simulink model "NBMS_App_Harness1"  (R2026b)
(part 3 of 4)

      AppIn_G3CommonFlt = false;
      state step_4_1
        AppIn_PMosfetfb = true;
      state step_4_2
        AppIn_HVMosfetfb = true;
      state step_4_3
        AppIn_DCDCMosfetfb = true;
      state step_4_4
        AppIn_PMosfetfb = false;
      (default) -> SleepToDischgToFlt2.step_4.step_4_1
      SleepToDischgToFlt2.step_4.step_4_1 -> SleepToDischgToFlt2.step_4.step_4_2 : [
          | after(0.2,sec)
          | ]
      SleepToDischgToFlt2.step_4.step_4_2 -> SleepToDischgToFlt2.step_4.step_4_3 : [
          | after(0.2,sec)
          | ]
      SleepToDischgToFlt2.step_4.step_4_3 -> SleepToDischgToFlt2.step_4.step_4_4 : [
          | after(0.2,sec)
          | ]
    state step_5
      AppIn_HardwiredIgn = false;
      state step_5_1
        AppIn_HVMosfetfb = false;
      (default) -> SleepToDischgToFlt2.step_5.step_5_1
    SleepToDischgToFlt2.step_6 -> SleepToDischgToFlt2.step_4 : [
        | after(0.2,sec)
        | ]
    (default) -> SleepToDischgToFlt2.Run
    SleepToDischgToFlt2.Run -> SleepToDischgToFlt2.step_1
    SleepToDischgToFlt2.step_1 -> SleepToDischgToFlt2.step_2 : [
        | after(0.2,sec)
        | ]
    SleepToDischgToFlt2.step_2 -> SleepToDischgToFlt2.step_3 : [
        | after(2,sec)
        | ]
    SleepToDischgToFlt2.step_3 -> SleepToDischgToFlt2.step_6 : [
        | after(6,sec)
        | ]
    SleepToDischgToFlt2.step_4 -> SleepToDischgToFlt2.step_5 : [
        | after(2,sec)
        | ]
  state SleepToDischgToFlt3
    state Run
      %% Initialize data outputs.
      AppIn_HardwiredIgn = false;
      AppIn_OBCwakeup = OBC_E.Sleep;
      AppIn_RTCwakeup = false;
      AppIn_MCUHVIL = false;
      AppIn_OBCHVIL = false;
      AppIn_SoCLEDSW = false;
      AppIn_ChgMode = Charger_Mode_E.OFF;
      AppIn_CVmodeTimer = CV_Mode_Timer_E.Off;
      AppIn_TRerror = false;
      AppIn_TRtimer = false;
      AppIn_G3CommonFlt = false;
      AppIn_G3DischargeFlt = false;
      AppIn_G4T1DischargeFlt = false;
      AppIn_G4T2DischargeFlt = false;
      AppIn_G4CommonFlt = false;
      AppIn_G4ChargeFlt = false;
      AppIn_OBCHeartbeatFail = false;
      AppIn_LoadVolt = 63;
      AppIn_PackVolt = 64;
      AppIn_ActiveDischg = Active_DisChrg_E.Inactive;
      AppIn_BattTemp = [26; 26; 26; 26; 26; 26;];
      AppIn_BattCurrent = 0;
      AppIn_BattVoltages = [4.2; 4.2; 4.2; 4.2; 4.2; 4.2; 4.2; 4.2; 4.2; 4.2; 4.2; 4.2; 4.2; 4.2; 4.2; 4.2; 4.2; 4.2; 4.2; 4.2];
      AppIn_LastStoredSOC = 0;
      AppIn_LastStoredCycle = 0;
      AppIn_I2Cerror = false;
      AppIn_LastStoredSOH = 0;
      AppIn_MachineStatus = VDU_MACHINE_STS_E.VDU_SLEEP;
      AppIn_HVMosfetfb = false;
      AppIn_DCDCMosfetfb = false;
      AppIn_PMosfetfb = false;
      AppIn_BMSVltSnsrFail = false;
      AppIn_BattPackTempSnsrFail = false;
      AppIn_VltImbFlt = false;
      AppIn_TempImbWarn = false;
      AppIn_EEPROMSoCWarn15 = false;
    state step_1
      AppIn_HardwiredIgn = true;
    state step_2
      AppIn_MCUHVIL = true;
      state step_2_1
        AppIn_PMosfetfb = true;
      state step_2_2
        AppIn_HVMosfetfb = true;
      state step_2_3
        AppIn_DCDCMosfetfb = true;
      state step_2_4
        AppIn_PMosfetfb = false;
      (default) -> SleepToDischgToFlt3.step_2.step_2_1
      SleepToDischgToFlt3.step_2.step_2_1 -> SleepToDischgToFlt3.step_2.step_2_2 : [
          | after(0.2,sec)
          | ]
      SleepToDischgToFlt3.step_2.step_2_2 -> SleepToDischgToFlt3.step_2.step_2_3 : [
          | after(0.2,sec)
          | ]
      SleepToDischgToFlt3.step_2.step_2_3 -> SleepToDischgToFlt3.step_2.step_2_4 : [
          | after(0.2,sec)
          | ]
    state step_3
      AppIn_G4CommonFlt = true;
    state step_6
      AppIn_OBCHVIL = true;
    state step_4
      AppIn_OBCHVIL = false;
      AppIn_G4CommonFlt = false;
      state step_4_1
        AppIn_PMosfetfb = true;
      state step_4_2
        AppIn_HVMosfetfb = true;
      state step_4_3
        AppIn_DCDCMosfetfb = true;
      state step_4_4
        AppIn_PMosfetfb = false;
      (default) -> SleepToDischgToFlt3.step_4.step_4_1
      SleepToDischgToFlt3.step_4.step_4_1 -> SleepToDischgToFlt3.step_4.step_4_2 : [
          | after(0.2,sec)
          | ]
      SleepToDischgToFlt3.step_4.step_4_2 -> SleepToDischgToFlt3.step_4.step_4_3 : [
          | after(0.2,sec)
          | ]
      SleepToDischgToFlt3.step_4.step_4_3 -> SleepToDischgToFlt3.step_4.step_4_4 : [
          | after(0.2,sec)
          | ]
    state step_5
      AppIn_HardwiredIgn = false;
      state step_5_1
        AppIn_HVMosfetfb = false;
      (default) -> SleepToDischgToFlt3.step_5.step_5_1
    (default) -> SleepToDischgToFlt3.Run
    SleepToDischgToFlt3.Run -> SleepToDischgToFlt3.step_1
    SleepToDischgToFlt3.step_1 -> SleepToDischgToFlt3.step_2 : [
        | after(0.2,sec)
        | ]
    SleepToDischgToFlt3.step_2 -> SleepToDischgToFlt3.step_3 : [
        | after(2,sec)
        | ]
    SleepToDischgToFlt3.step_3 -> SleepToDischgToFlt3.step_6 : [
        | after(6,sec)
        | ]
    SleepToDischgToFlt3.step_6 -> SleepToDischgToFlt3.step_4 : [
        | after(0.2,sec)
        | ]
    SleepToDischgToFlt3.step_4 -> SleepToDischgToFlt3.step_5 : [
        | after(2,sec)
        | ]
  state SleepToChgToFlt
    state Run
      %% Initialize data outputs.
      AppIn_HardwiredIgn = false;
      AppIn_OBCwakeup = OBC_E.Sleep;
      AppIn_RTCwakeup = false;
      AppIn_MCUHVIL = false;
      AppIn_OBCHVIL = false;
      AppIn_SoCLEDSW = false;
      AppIn_ChgMode = Charger_Mode_E.OFF;
      AppIn_CVmodeTimer = CV_Mode_Timer_E.Off;
      AppIn_TRerror = false;
      AppIn_TRtimer = false;
      AppIn_G3CommonFlt = false;
      AppIn_G3DischargeFlt = false;
      AppIn_G4T1DischargeFlt = false;
      AppIn_G4T2DischargeFlt = false;
      AppIn_G4CommonFlt = false;
      AppIn_G4ChargeFlt = false;
      AppIn_OBCHeartbeatFail = false;
      AppIn_LoadVolt = 63;
      AppIn_PackVolt = 64;
      AppIn_ActiveDischg = Active_DisChrg_E.Inactive;
      AppIn_BattTemp = [26; 26; 26; 26; 26; 26;];
      AppIn_BattCurrent = 0;
      AppIn_BattVoltages = [4.2; 4.2; 4.2; 4.2; 4.2; 4.2; 4.2; 4.2; 4.2; 4.2; 4.2; 4.2; 4.2; 4.2; 4.2; 4.2; 4.2; 4.2; 4.2; 4.2];
      AppIn_LastStoredSOC = 0;
      AppIn_LastStoredCycle = 0;
      AppIn_I2Cerror = false;
      AppIn_LastStoredSOH = 0;
      AppIn_MachineStatus = VDU_MACHINE_STS_E.VDU_SLEEP;
      AppIn_HVMosfetfb = false;
      AppIn_DCDCMosfetfb = false;
      AppIn_PMosfetfb = false;
      AppIn_BMSVltSnsrFail = false;
      AppIn_BattPackTempSnsrFail = false;
      AppIn_VltImbFlt = false;
      AppIn_TempImbWarn = false;
      AppIn_EEPROMSoCWarn15 = false;
    state step_1
      AppIn_OBCwakeup = OBC_E.Wake_Up;
      AppIn_OBCHVIL = true;
    state step_2
      state step_2_1
        AppIn_PMosfetfb = true;
      state step_2_2
        AppIn_HVMosfetfb = true;
      state step_2_3
        AppIn_PMosfetfb = false;
      (default) -> SleepToChgToFlt.step_2.step_2_1
      SleepToChgToFlt.step_2.step_2_1 -> SleepToChgToFlt.step_2.step_2_2 : [
          | after(0.3,sec)
          | ]
      SleepToChgToFlt.step_2.step_2_2 -> SleepToChgToFlt.step_2.step_2_3 : [
          | after(0.5,sec)
          | ]
    state step_3
      AppIn_G3CommonFlt = true;
    state step_4
      state step_4_1
        AppIn_ChgMode = Charger_Mode_E.Error;
      state step_4_2
        AppIn_ChgMode = Charger_Mode_E.OFF;
      (default) -> SleepToChgToFlt.step_4.step_4_1
      SleepToChgToFlt.step_4.step_4_1 -> SleepToChgToFlt.step_4.step_4_2 : [
          | after(0.1,sec)
          | ]
    state step_5
      AppIn_G3CommonFlt = false;
    state step_6
      AppIn_OBCHVIL = false;
      AppIn_OBCwakeup = OBC_E.Sleep;
      state step_6_1
        AppIn_HVMosfetfb = false;
      (default) -> SleepToChgToFlt.step_6.step_6_1
    (default) -> SleepToChgToFlt.Run
    SleepToChgToFlt.Run -> SleepToChgToFlt.step_1 : [
        | after(0.2,sec)
        | ]
    SleepToChgToFlt.step_1 -> SleepToChgToFlt.step_2 : [
        | after(0.2,sec)
        | ]
    SleepToChgToFlt.step_2 -> SleepToChgToFlt.step_3 : [
        | after(2,sec)
        | ]
    SleepToChgToFlt.step_3 -> SleepToChgToFlt.step_4 : [
        | after(1,sec)
        | ]
    SleepToChgToFlt.step_4 -> SleepToChgToFlt.step_5 : [
        | after(1,sec)
        | ]
    SleepToChgToFlt.step_5 -> SleepToChgToFlt.step_6 : [
        | after(2,sec)
        | ]
  state SleepToChgToFltToDischg
    state Run
      %% Initialize data outputs.
      AppIn_HardwiredIgn = false;
      AppIn_OBCwakeup = OBC_E.Sleep;
      AppIn_RTCwakeup = false;
      AppIn_MCUHVIL = false;
      AppIn_OBCHVIL = false;
      AppIn_SoCLEDSW = false;
      AppIn_ChgMode = Charger_Mode_E.OFF;
      AppIn_CVmodeTimer = CV_Mode_Timer_E.Off;
      AppIn_TRerror = false;
      AppIn_TRtimer = false;
      AppIn_G3CommonFlt = false;
      AppIn_G3DischargeFlt = false;
      AppIn_G4T1DischargeFlt = false;
      AppIn_G4T2DischargeFlt = false;
      AppIn_G4CommonFlt = false;
      AppIn_G4ChargeFlt = false;
      AppIn_OBCHeartbeatFail = false;
      AppIn_LoadVolt = 63;
      AppIn_PackVolt = 64;
      AppIn_ActiveDischg = Active_DisChrg_E.Inactive;
      AppIn_BattTemp = [26; 26; 26; 26; 26; 26;];
      AppIn_BattCurrent = 0;
      AppIn_BattVoltages = [4.2; 4.2; 4.2; 4.2; 4.2; 4.2; 4.2; 4.2; 4.2; 4.2; 4.2; 4.2; 4.2; 4.2; 4.2; 4.2; 4.2; 4.2; 4.2; 4.2];
      AppIn_LastStoredSOC = 0;
      AppIn_LastStoredCycle = 0;
      AppIn_I2Cerror = false;
      AppIn_LastStoredSOH = 0;
      AppIn_MachineStatus = VDU_MACHINE_STS_E.VDU_SLEEP;
      AppIn_HVMosfetfb = false;
      AppIn_DCDCMosfetfb = false;
      AppIn_PMosfetfb = false;
      AppIn_BMSVltSnsrFail = false;
      AppIn_BattPackTempSnsrFail = false;
      AppIn_VltImbFlt = false;
      AppIn_TempImbWarn = false;
      AppIn_EEPROMSoCWarn15 = false;
    state step_1
      AppIn_OBCwakeup = OBC_E.Wake_Up;
      AppIn_OBCHVIL = true;
    state step_2
      state step_2_1
        AppIn_PMosfetfb = true;
      state step_2_2
        AppIn_HVMosfetfb = true;
      state step_2_3
        AppIn_PMosfetfb = false;
      (default) -> SleepToChgToFltToDischg.step_2.step_2_1
      SleepToChgToFltToDischg.step_2.step_2_1 -> SleepToChgToFltToDischg.step_2.step_2_2 : [
          | after(0.3,sec)
          | ]
      SleepToChgToFltToDischg.step_2.step_2_2 -> SleepToChgToFltToDischg.step_2.step_2_3 : [
          | after(0.5,sec)
          | ]
    state step_3
      AppIn_G4ChargeFlt= true;
    state step_4
      AppIn_OBCHVIL = false;
      AppIn_OBCwakeup = OBC_E.Sleep;
      AppIn_HardwiredIgn = true;
      AppIn_MCUHVIL = true;
      state step_4_1
        AppIn_PMosfetfb = true;
      state step_4_2
        AppIn_HVMosfetfb = true;
      state step_4_3
        AppIn_DCDCMosfetfb = true;
      state step_4_4
        AppIn_PMosfetfb = false;
      (default) -> SleepToChgToFltToDischg.step_4.step_4_1
      SleepToChgToFltToDischg.step_4.step_4_1 -> SleepToChgToFltToDischg.step_4.step_4_2 : [
          | after(0.3,sec)
          | ]
      SleepToChgToFltToDischg.step_4.step_4_2 -> SleepToChgToFltToDischg.step_4.step_4_3 : [
          | after(0.2,sec)
          | ]
      SleepToChgToFltToDischg.step_4.step_4_3 -> SleepToChgToFltToDischg.step_4.step_4_4 : [
          | after(0.2,sec)
          | ]
    state step_5
      AppIn_HardwiredIgn = false;
      state step_6_1
        AppIn_HVMosfetfb = false;
      (default) -> SleepToChgToFltToDischg.step_5.step_6_1
    (default) -> SleepToChgToFltToDischg.Run
    SleepToChgToFltToDischg.Run -> SleepToChgToFltToDischg.step_1 : [
        | after(0.2,sec)
        | ]
    SleepToChgToFltToDischg.step_1 -> SleepToChgToFltToDischg.step_2 : [
        | after(0.2,sec)
        | ]
    SleepToChgToFltToDischg.step_2 -> SleepToChgToFltToDischg.step_3 : [
        | after(2,sec)
        | ]
    SleepToChgToFltToDischg.step_3 -> SleepToChgToFltToDischg.step_4 : [
        | after(1,sec)
        | ]
    SleepToChgToFltToDischg.step_4 -> SleepToChgToFltToDischg.step_5 : [
        | after(2,sec)
        | ]
  state SleepToChgToFltToDischg1
    state Run
      %% Initialize data outputs.
      AppIn_HardwiredIgn = false;
      AppIn_OBCwakeup = OBC_E.Sleep;
      AppIn_RTCwakeup = false;
      AppIn_MCUHVIL = false;
      AppIn_OBCHVIL = false;
      AppIn_SoCLEDSW = false;
      AppIn_ChgMode = Charger_Mode_E.OFF;
      AppIn_CVmodeTimer = CV_Mode_Timer_E.Off;
      AppIn_TRerror = false;
      AppIn_TRtimer = false;
      AppIn_G3CommonFlt = false;
      AppIn_G3DischargeFlt = false;
      AppIn_G4T1DischargeFlt = false;
      AppIn_G4T2DischargeFlt = false;
      AppIn_G4CommonFlt = false;
      AppIn_G4ChargeFlt = false;
      AppIn_OBCHeartbeatFail = false;
      AppIn_LoadVolt = 63;
      AppIn_PackVolt = 64;
      AppIn_ActiveDischg = Active_DisChrg_E.Inactive;
      AppIn_BattTemp = [26; 26; 26; 26; 26; 26;];
      AppIn_BattCurrent = 0;
      AppIn_BattVoltages = [4.2; 4.2; 4.2; 4.2; 4.2; 4.2; 4.2; 4.2; 4.2; 4.2; 4.2; 4.2; 4.2; 4.2; 4.2; 4.2; 4.2; 4.2; 4.2; 4.2];
      AppIn_LastStoredSOC = 0;
      AppIn_LastStoredCycle = 0;
      AppIn_I2Cerror = false;
      AppIn_LastStoredSOH = 0;
      AppIn_MachineStatus = VDU_MACHINE_STS_E.VDU_SLEEP;
      AppIn_HVMosfetfb = false;
      AppIn_DCDCMosfetfb = false;
      AppIn_PMosfetfb = false;
      AppIn_BMSVltSnsrFail = false;
      AppIn_BattPackTempSnsrFail = false;
      AppIn_VltImbFlt = false;
      AppIn_TempImbWarn = false;
      AppIn_EEPROMSoCWarn15 = false;
    state step_1
      AppIn_OBCwakeup = OBC_E.Wake_Up;
      AppIn_OBCHVIL = true;
    state step_2
      state step_2_1
        AppIn_PMosfetfb = true;
      state step_2_2
        AppIn_HVMosfetfb = true;
      state step_2_3
        AppIn_PMosfetfb = false;
      (default) -> SleepToChgToFltToDischg1.step_2.step_2_1
      SleepToChgToFltToDischg1.step_2.step_2_1 -> SleepToChgToFltToDischg1.step_2.step_2_2 : [
          | after(0.3,sec)
          | ]
      SleepToChgToFltToDischg1.step_2.step_2_2 -> SleepToChgToFltToDischg1.step_2.step_2_3 : [
          | after(0.5,sec)
          | ]
    state step_3
      AppIn_G4CommonFlt= true;
    state step_4
      AppIn_OBCHVIL = false;
      AppIn_OBCwakeup = OBC_E.Sleep;
      AppIn_HardwiredIgn = true;
      AppIn_MCUHVIL = true;
      AppIn_G4CommonFlt= false;
      state step_4_1
        AppIn_PMosfetfb = true;
      state step_4_2
        AppIn_HVMosfetfb = true;
      state step_4_3
        AppIn_DCDCMosfetfb = true;
      state step_4_4
        AppIn_PMosfetfb = false;
      (default) -> SleepToChgToFltToDischg1.step_4.step_4_1
      SleepToChgToFltToDischg1.step_4.step_4_1 -> SleepToChgToFltToDischg1.step_4.step_4_2 : [
          | after(0.3,sec)
          | ]
      SleepToChgToFltToDischg1.step_4.step_4_2 -> SleepToChgToFltToDischg1.step_4.step_4_3 : [
          | after(0.2,sec)
          | ]
      SleepToChgToFltToDischg1.step_4.step_4_3 -> SleepToChgToFltToDischg1.step_4.step_4_4 : [
          | after(0.2,sec)
          | ]
    state step_5
      AppIn_HardwiredIgn = false;
      state step_6_1
        AppIn_HVMosfetfb = false;
      (default) -> SleepToChgToFltToDischg1.step_5.step_6_1
    state step_6
      AppIn_G4CommonFlt= true;
    (default) -> SleepToChgToFltToDischg1.Run
    SleepToChgToFltToDischg1.Run -> SleepToChgToFltToDischg1.step_1 : [
        | after(0.2,sec)
        | ]
    SleepToChgToFltToDischg1.step_1 -> SleepToChgToFltToDischg1.step_2 : [
        | after(0.2,sec)
        | ]
    SleepToChgToFltToDischg1.step_2 -> SleepToChgToFltToDischg1.step_3 : [
        | after(2,sec)
        | ]
    SleepToChgToFltToDischg1.step_3 -> SleepToChgToFltToDischg1.step_4 : [
        | after(1,sec)
        | ]
    SleepToChgToFltToDischg1.step_4 -> SleepToChgToFltToDischg1.step_5 : [
        | after(2,sec)
        | ]
    SleepToChgToFltToDischg1.step_5 -> SleepToChgToFltToDischg1.step_6 : [
        | after(0.3,sec)
        | ]
  state SleepToDischgToFltToChg
    state Run
      %% Initialize data outputs.
      AppIn_HardwiredIgn = false;
      AppIn_OBCwakeup = OBC_E.Sleep;
      AppIn_RTCwakeup = false;
      AppIn_MCUHVIL = false;
      AppIn_OBCHVIL = false;
      AppIn_SoCLEDSW = false;
      AppIn_ChgMode = Charger_Mode_E.OFF;
      AppIn_CVmodeTimer = CV_Mode_Timer_E.Off;
      AppIn_TRerror = false;
      AppIn_TRtimer = false;
      AppIn_G3CommonFlt = false;
      AppIn_G3DischargeFlt = false;
      AppIn_G4T1DischargeFlt = false;
      AppIn_G4T2DischargeFlt = false;
      AppIn_G4CommonFlt = false;
      AppIn_G4ChargeFlt = false;
      AppIn_OBCHeartbeatFail = false;
      AppIn_LoadVolt = 63;
      AppIn_PackVolt = 64;
      AppIn_ActiveDischg = Active_DisChrg_E.Inactive;
      AppIn_BattTemp = [26; 26; 26; 26; 26; 26;];
      AppIn_BattCurrent = 0;
      AppIn_BattVoltages = [4.2; 4.2; 4.2; 4.2; 4.2; 4.2; 4.2; 4.2; 4.2; 4.2; 4.2; 4.2; 4.2; 4.2; 4.2; 4.2; 4.2; 4.2; 4.2; 4.2];
      AppIn_LastStoredSOC = 0;
      AppIn_LastStoredCycle = 0;
      AppIn_I2Cerror = false;
      AppIn_LastStoredSOH = 0;
      AppIn_MachineStatus = VDU_MACHINE_STS_E.VDU_SLEEP;
      AppIn_HVMosfetfb = false;
      AppIn_DCDCMosfetfb = false;
      AppIn_PMosfetfb = false;
      AppIn_BMSVltSnsrFail = false;
      AppIn_BattPackTempSnsrFail = false;
      AppIn_VltImbFlt = false;
      AppIn_TempImbWarn = false;
      AppIn_EEPROMSoCWarn15 = false;
    state step_1
      AppIn_HardwiredIgn = true;
      AppIn_MCUHVIL = true;
    state step_2
      state step_2_1
        AppIn_PMosfetfb = true;
      state step_2_2
        AppIn_HVMosfetfb = true;
      state step_2_4
        AppIn_DCDCMosfetfb = true;
      state step_2_3
        AppIn_PMosfetfb = false;
      (default) -> SleepToDischgToFltToChg.step_2.step_2_1
      SleepToDischgToFltToChg.step_2.step_2_1 -> SleepToDischgToFltToChg.step_2.step_2_2 : [
          | after(0.3,sec)
          | ]
      SleepToDischgToFltToChg.step_2.step_2_2 -> SleepToDischgToFltToChg.step_2.step_2_4 : [
          | after(0.2,sec)
          | ]
      SleepToDischgToFltToChg.step_2.step_2_4 -> SleepToDischgToFltToChg.step_2.step_2_3 : [
          | after(0.2,sec)
          | ]
    state step_3
      AppIn_G4T1DischargeFlt= true;
    state step_4
      AppIn_OBCHVIL = true;
      AppIn_OBCwakeup = OBC_E.Wake_Up;
      state step_4_1
        AppIn_PMosfetfb = true;
      state step_4_2
        AppIn_HVMosfetfb = true;
      state step_4_3
        AppIn_DCDCMosfetfb = true;
      state step_4_4
        AppIn_PMosfetfb = false;
      (default) -> SleepToDischgToFltToChg.step_4.step_4_1
      SleepToDischgToFltToChg.step_4.step_4_1 -> SleepToDischgToFltToChg.step_4.step_4_2 : [
          | after(0.3,sec)
          | ]
      SleepToDischgToFltToChg.step_4.step_4_2 -> SleepToDischgToFltToChg.step_4.step_4_3 : [
          | after(0.2,sec)
          | ]
      SleepToDischgToFltToChg.step_4.step_4_3 -> SleepToDischgToFltToChg.step_4.step_4_4 : [
          | after(0.2,sec)
          | ]
    state step_5
      AppIn_HardwiredIgn = false;
      AppIn_OBCHVIL = false;
      AppIn_OBCwakeup = OBC_E.Sleep;
      state step_6_1
        AppIn_HVMosfetfb = false;
      (default) -> SleepToDischgToFltToChg.step_5.step_6_1
    (default) -> SleepToDischgToFltToChg.Run
    SleepToDischgToFltToChg.Run -> SleepToDischgToFltToChg.step_1 : [
        | after(0.2,sec)
        | ]
    SleepToDischgToFltToChg.step_1 -> SleepToDischgToFltToChg.step_2 : [
        | after(0.2,sec)
        | ]
    SleepToDischgToFltToChg.step_2 -> SleepToDischgToFltToChg.step_3 : [
        | after(2,sec)
        | ]
    SleepToDischgToFltToChg.step_3 -> SleepToDischgToFltToChg.step_4 : [
        | after(1,sec)
        | ]
    SleepToDischgToFltToChg.step_4 -> SleepToDischgToFltToChg.step_5 : [
        | after(2,sec)
        | ]
  state SleepToDischgToFltToChg1
    state Run
      %% Initialize data outputs.
      AppIn_HardwiredIgn = false;
      AppIn_OBCwakeup = OBC_E.Sleep;
      AppIn_RTCwakeup = false;
      AppIn_MCUHVIL = false;
      AppIn_OBCHVIL = false;
      AppIn_SoCLEDSW = false;
      AppIn_ChgMode = Charger_Mode_E.OFF;
      AppIn_CVmodeTimer = CV_Mode_Timer_E.Off;
      AppIn_TRerror = false;
      AppIn_TRtimer = false;
      AppIn_G3CommonFlt = false;
      AppIn_G3DischargeFlt = false;
      AppIn_G4T1DischargeFlt = false;
      AppIn_G4T2DischargeFlt = false;
      AppIn_G4CommonFlt = false;
      AppIn_G4ChargeFlt = false;
      AppIn_OBCHeartbeatFail = false;
      AppIn_LoadVolt = 63;
      AppIn_PackVolt = 64;
      AppIn_ActiveDischg = Active_DisChrg_E.Inactive;
      AppIn_BattTemp = [26; 26; 26; 26; 26; 26;];
      AppIn_BattCurrent = 0;
      AppIn_BattVoltages = [4.2; 4.2; 4.2; 4.2; 4.2; 4.2; 4.2; 4.2; 4.2; 4.2; 4.2; 4.2; 4.2; 4.2; 4.2; 4.2; 4.2; 4.2; 4.2; 4.2];
      AppIn_LastStoredSOC = 0;
      AppIn_LastStoredCycle = 0;
      AppIn_I2Cerror = false;
      AppIn_LastStoredSOH = 0;
      AppIn_MachineStatus = VDU_MACHINE_STS_E.VDU_SLEEP;
      AppIn_HVMosfetfb = false;
      AppIn_DCDCMosfetfb = false;
      AppIn_PMosfetfb = false;
      AppIn_BMSVltSnsrFail = false;
      AppIn_BattPackTempSnsrFail = false;
      AppIn_VltImbFlt = false;
      AppIn_TempImbWarn = false;
      AppIn_EEPROMSoCWarn15 = false;
    state step_1
      AppIn_HardwiredIgn = true;
      AppIn_MCUHVIL = true;
    state step_2
      state step_2_1
        AppIn_PMosfetfb = true;
      state step_2_2
        AppIn_HVMosfetfb = true;
      state step_2_4
        AppIn_DCDCMosfetfb = true;
      state step_2_3
        AppIn_PMosfetfb = false;
      (default) -> SleepToDischgToFltToChg1.step_2.step_2_1
      SleepToDischgToFltToChg1.step_2.step_2_1 -> SleepToDischgToFltToChg1.step_2.step_2_2 : [
          | after(0.3,sec)
          | ]
      SleepToDischgToFltToChg1.step_2.step_2_2 -> SleepToDischgToFltToChg1.step_2.step_2_4 : [
          | after(0.2,sec)
          | ]
      SleepToDischgToFltToChg1.step_2.step_2_4 -> SleepToDischgToFltToChg1.step_2.step_2_3 : [
          | after(0.2,sec)
          | ]
    state step_3
      AppIn_G3DischargeFlt= true;
    state step_4
      AppIn_OBCHVIL = true;
      AppIn_OBCwakeup = OBC_E.Wake_Up;
      state step_4_1
        AppIn_PMosfetfb = true;
      state step_4_2
        AppIn_HVMosfetfb = true;
      state step_4_3
        AppIn_DCDCMosfetfb = true;
      state step_4_4
        AppIn_PMosfetfb = false;
      (default) -> SleepToDischgToFltToChg1.step_4.step_4_1
      SleepToDischgToFltToChg1.step_4.step_4_1 -> SleepToDischgToFltToChg1.step_4.step_4_2 : [
          | after(0.3,sec)
          | ]
      SleepToDischgToFltToChg1.step_4.step_4_2 -> SleepToDischgToFltToChg1.step_4.step_4_3 : [
          | after(0.2,sec)
          | ]
      SleepToDischgToFltToChg1.step_4.step_4_3 -> SleepToDischgToFltToChg1.step_4.step_4_4 : [
          | after(0.2,sec)
          | ]
    state step_5
      AppIn_HardwiredIgn = false;
      AppIn_OBCHVIL = false;
      AppIn_OBCwakeup = OBC_E.Sleep;
      state step_6_1
        AppIn_HVMosfetfb = false;
      (default) -> SleepToDischgToFltToChg1.step_5.step_6_1
    (default) -> SleepToDischgToFltToChg1.Run
    SleepToDischgToFltToChg1.Run -> SleepToDischgToFltToChg1.step_1 : [
        | after(0.2,sec)
        | ]
    SleepToDischgToFltToChg1.step_1 -> SleepToDischgToFltToChg1.step_2 : [
        | after(0.2,sec)
        | ]
    SleepToDischgToFltToChg1.step_2 -> SleepToDischgToFltToChg1.step_3 : [
        | after(2,sec)
        | ]
    SleepToDischgToFltToChg1.step_3 -> SleepToDischgToFltToChg1.step_4 : [
        | after(1,sec)
        | ]
    SleepToDischgToFltToChg1.step_4 -> SleepToDischgToFltToChg1.step_5 : [
        | after(2,sec)
        | ]
  state SleepToDischgToFltToChg2
    state Run
      %% Initialize data outputs.
      AppIn_HardwiredIgn = false;
      AppIn_OBCwakeup = OBC_E.Sleep;
      AppIn_RTCwakeup = false;
      AppIn_MCUHVIL = false;
      AppIn_OBCHVIL = false;
      AppIn_SoCLEDSW = false;
      AppIn_ChgMode = Charger_Mode_E.OFF;
      AppIn_CVmodeTimer = CV_Mode_Timer_E.Off;
      AppIn_TRerror = false;
      AppIn_TRtimer = false;
      AppIn_G3CommonFlt = false;
      AppIn_G3DischargeFlt = false;
      AppIn_G4T1DischargeFlt = false;
      AppIn_G4T2DischargeFlt = false;
      AppIn_G4CommonFlt = false;
      AppIn_G4ChargeFlt = false;
      AppIn_OBCHeartbeatFail = false;
      AppIn_LoadVolt = 63;
      AppIn_PackVolt = 64;
      AppIn_ActiveDischg = Active_DisChrg_E.Inactive;
      AppIn_BattTemp = [26; 26; 26; 26; 26; 26;];
      AppIn_BattCurrent = 0;
      AppIn_BattVoltages = [4.2; 4.2; 4.2; 4.2; 4.2; 4.2; 4.2; 4.2; 4.2; 4.2; 4.2; 4.2; 4.2; 4.2; 4.2; 4.2; 4.2; 4.2; 4.2; 4.2];
      AppIn_LastStoredSOC = 0;
      AppIn_LastStoredCycle = 0;
      AppIn_I2Cerror = false;
      AppIn_LastStoredSOH = 0;
      AppIn_MachineStatus = VDU_MACHINE_STS_E.VDU_SLEEP;
      AppIn_HVMosfetfb = false;
      AppIn_DCDCMosfetfb = false;
      AppIn_PMosfetfb = false;
      AppIn_BMSVltSnsrFail = false;
      AppIn_BattPackTempSnsrFail = false;
      AppIn_VltImbFlt = false;
      AppIn_TempImbWarn = false;
      AppIn_EEPROMSoCWarn15 = false;
    state step_1
      AppIn_HardwiredIgn = true;
      AppIn_MCUHVIL = true;
    state step_2
      state step_2_1
        AppIn_PMosfetfb = true;
      state step_2_2
        AppIn_HVMosfetfb = true;
      state step_2_4
        AppIn_DCDCMosfetfb = true;
      state step_2_3
        AppIn_PMosfetfb = false;
      (default) -> SleepToDischgToFltToChg2.step_2.step_2_1
      SleepToDischgToFltToChg2.step_2.step_2_1 -> SleepToDischgToFltToChg2.step_2.step_2_2 : [
          | after(0.3,sec)
          | ]
      SleepToDischgToFltToChg2.step_2.step_2_2 -> SleepToDischgToFltToChg2.step_2.step_2_4 : [
          | after(0.2,sec)
          | ]
      SleepToDischgToFltToChg2.step_2.step_2_4 -> SleepToDischgToFltToChg2.step_2.step_2_3 : [
          | after(0.2,sec)
          | ]
    state step_3
      AppIn_G4T2DischargeFlt= true;
    state step_4
      AppIn_OBCHVIL = true;
      AppIn_OBCwakeup = OBC_E.Wake_Up;
      state step_4_1
        AppIn_PMosfetfb = true;
      state step_4_2
        AppIn_HVMosfetfb = true;
      state step_4_3
        AppIn_DCDCMosfetfb = true;
      state step_4_4
        AppIn_PMosfetfb = false;
      (default) -> SleepToDischgToFltToChg2.step_4.step_4_1
      SleepToDischgToFltToChg2.step_4.step_4_1 -> SleepToDischgToFltToChg2.step_4.step_4_2 : [
          | after(0.3,sec)
          | ]
      SleepToDischgToFltToChg2.step_4.step_4_2 -> SleepToDischgToFltToChg2.step_4.step_4_3 : [
          | after(0.2,sec)
          | ]
      SleepToDischgToFltToChg2.step_4.step_4_3 -> SleepToDischgToFltToChg2.step_4.step_4_4 : [
          | after(0.2,sec)
          | ]
    state step_5
      AppIn_HardwiredIgn = false;
      AppIn_OBCHVIL = false;
      AppIn_OBCwakeup = OBC_E.Sleep;
      state step_6_1
        AppIn_HVMosfetfb = false;
      (default) -> SleepToDischgToFltToChg2.step_5.step_6_1
    (default) -> SleepToDischgToFltToChg2.Run
    SleepToDischgToFltToChg2.Run -> SleepToDischgToFltToChg2.step_1 : [
        | after(0.2,sec)
        | ]
    SleepToDischgToFltToChg2.step_1 -> SleepToDischgToFltToChg2.step_2 : [
        | after(0.2,sec)
        | ]
    SleepToDischgToFltToChg2.step_2 -> SleepToDischgToFltToChg2.step_3 : [
        | after(2,sec)
        | ]
    SleepToDischgToFltToChg2.step_3 -> SleepToDischgToFltToChg2.step_4 : [
        | after(1,sec)
        | ]
    SleepToDischgToFltToChg2.step_4 -> SleepToDischgToFltToChg2.step_5 : [
        | after(2,sec)
        | ]
  state ChargingSequence
    state Run
      %% Initialize data outputs.
      AppIn_HardwiredIgn = false;
      AppIn_OBCwakeup = OBC_E.Sleep;
      AppIn_RTCwakeup = false;
      AppIn_MCUHVIL = false;
      AppIn_OBCHVIL = false;
      AppIn_SoCLEDSW = false;
      AppIn_ChgMode = Charger_Mode_E.OFF;
      AppIn_CVmodeTimer = CV_Mode_Timer_E.Off;
      AppIn_TRerror = false;
      AppIn_TRtimer = false;
      AppIn_G3CommonFlt = false;
      AppIn_G3DischargeFlt = false;
      AppIn_G4T1DischargeFlt = false;
      AppIn_G4T2DischargeFlt = false;
      AppIn_G4CommonFlt = false;
      AppIn_G4ChargeFlt = false;
      AppIn_OBCHeartbeatFail = false;
      AppIn_LoadVolt = 78;
      AppIn_PackVolt = 74;
      AppIn_ActiveDischg = Active_DisChrg_E.Inactive;
      AppIn_BattTemp = [26; 26; 26; 26; 26; 26;];
      AppIn_BattCurrent = 0;
      AppIn_BattVoltages = [4.41; 4.41; 4.41; 4.41; 4.41; 4.41; 4.41; 4.41; 4.41; 4.41; 4.41; 4.41; 4.41; 4.41; 4.41; 4.41; 4.41; 4.41; 4.41; 3.2];
      AppIn_LastStoredSOC = 0;
      AppIn_LastStoredCycle = 0;
      AppIn_I2Cerror = false;
      AppIn_LastStoredSOH = 0;
      AppIn_MachineStatus = VDU_MACHINE_STS_E.VDU_SLEEP;
      AppIn_HVMosfetfb = false;
      AppIn_DCDCMosfetfb = false;
      AppIn_PMosfetfb = false;
      AppIn_BMSVltSnsrFail = false;
      AppIn_BattPackTempSnsrFail = false;
      AppIn_VltImbFlt = false;
      AppIn_TempImbWarn = false;
      AppIn_EEPROMSoCWarn15 = false;
    state step_1
      AppIn_OBCwakeup = OBC_E.Wake_Up;
      AppIn_OBCHVIL = true;
    state step_2
      state step_2_1
        AppIn_PMosfetfb = true;
      state step_2_2
        AppIn_HVMosfetfb = true;
      state step_2_3
        AppIn_PMosfetfb = false;
      (default) -> ChargingSequence.step_2.step_2_1
      ChargingSequence.step_2.step_2_1 -> ChargingSequence.step_2.step_2_2 : [
          | after(0.3,sec)
          | ]
      ChargingSequence.step_2.step_2_2 -> ChargingSequence.step_2.step_2_3 : [
          | after(0.5,sec)
          | ]
    state step_4
      AppIn_OBCwakeup = OBC_E.Sleep;
      AppIn_HVMosfetfb = false;
    (default) -> ChargingSequence.Run
    ChargingSequence.Run -> ChargingSequence.step_1 : [
        | after(0.1,sec)
        | ]
    ChargingSequence.step_1 -> ChargingSequence.step_2 : [
        | after(0.2,sec)
        | ]
    ChargingSequence.step_2 -> ChargingSequence.step_4 : [
        | after(6,sec)
        | ]
  state ChargeSeq
    state Run
      %% Initialize data outputs.
      AppIn_HardwiredIgn = false;
      AppIn_OBCwakeup = OBC_E.Sleep;
      AppIn_RTCwakeup = false;
      AppIn_MCUHVIL = false;
      AppIn_OBCHVIL = false;
      AppIn_SoCLEDSW = false;
      AppIn_ChgMode = Charger_Mode_E.OFF;
      AppIn_CVmodeTimer = CV_Mode_Timer_E.Off;
      AppIn_TRerror = false;
      AppIn_TRtimer = false;
      AppIn_G3CommonFlt = false;
      AppIn_G3DischargeFlt = false;
      AppIn_G4T1DischargeFlt = false;
      AppIn_G4T2DischargeFlt = false;
      AppIn_G4CommonFlt = false;
      AppIn_G4ChargeFlt = false;
      AppIn_OBCHeartbeatFail = false;
      AppIn_LoadVolt = 80;
      AppIn_PackVolt = 78;
      AppIn_ActiveDischg = Active_DisChrg_E.Inactive;
      AppIn_BattTemp = [26; 26; 26; 26; 26; 26;];
      AppIn_BattCurrent = 0;
      AppIn_BattVoltages = [4.41; 4.41; 4.41; 4.41; 4.41; 4.41; 4.41; 4.41; 4.41; 4.41; 4.41; 4.41; 4.41; 4.41; 4.41; 4.41; 4.41; 4.41; 4.41; 3.2];
      AppIn_LastStoredSOC = 0;
      AppIn_LastStoredCycle = 0;
      AppIn_I2Cerror = false;
      AppIn_LastStoredSOH = 0;
      AppIn_MachineStatus = VDU_MACHINE_STS_E.VDU_SLEEP;
      AppIn_HVMosfetfb = false;
      AppIn_DCDCMosfetfb = false;
      AppIn_PMosfetfb = false;
      AppIn_BMSVltSnsrFail = false;
      AppIn_BattPackTempSnsrFail = false;
      AppIn_VltImbFlt = false;
      AppIn_TempImbWarn = false;
      AppIn_EEPROMSoCWarn15 = false;
    state step_1
      AppIn_OBCwakeup = OBC_E.Wake_Up;
      AppIn_OBCHVIL = true;
    state step_2
      state step_2_1
        AppIn_PMosfetfb = true;
      state step_2_2
        AppIn_HVMosfetfb = true;
      state step_2_3
        AppIn_PMosfetfb = false;
      (default) -> ChargeSeq.step_2.step_2_1
      ChargeSeq.step_2.step_2_1 -> ChargeSeq.step_2.step_2_2 : [
          | after(0.3,sec)
          | ]
      ChargeSeq.step_2.step_2_2 -> ChargeSeq.step_2.step_2_3 : [
          | after(0.5,sec)
          | ]
    state step_4
      AppIn_HVMosfetfb = false;
    (default) -> ChargeSeq.Run
    ChargeSeq.Run -> ChargeSeq.step_1 : [
        | after(0.1,sec)
        | ]
    ChargeSeq.step_1 -> ChargeSeq.step_2 : [
        | after(0.2,sec)
        | ]
    ChargeSeq.step_2 -> ChargeSeq.step_4 : [
        | after(20,sec)
        | ]
  state ChargeSeqG2Fault
    state Run
      %% Initialize data outputs.
      AppIn_HardwiredIgn = false;
      AppIn_OBCwakeup = OBC_E.Sleep;
      AppIn_RTCwakeup = false;
      AppIn_MCUHVIL = false;
      AppIn_OBCHVIL = false;
      AppIn_SoCLEDSW = false;
      AppIn_ChgMode = Charger_Mode_E.OFF;
      AppIn_CVmodeTimer = CV_Mode_Timer_E.Off;
      AppIn_TRerror = false;
      AppIn_TRtimer = false;
      AppIn_G3CommonFlt = false;
      AppIn_G3DischargeFlt = false;
      AppIn_G4T1DischargeFlt = false;
      AppIn_G4T2DischargeFlt = false;
      AppIn_G4CommonFlt = false;
      AppIn_G4ChargeFlt = false;
      AppIn_OBCHeartbeatFail = false;
      AppIn_LoadVolt = 80;
      AppIn_PackVolt = 78;
      AppIn_ActiveDischg = Active_DisChrg_E.Inactive;
      AppIn_BattTemp = [26; 26; 26; 26; 26; 26;];
      AppIn_BattCurrent = 0;
      AppIn_BattVoltages = [4.41; 4.41; 4.41; 4.41; 4.41; 4.41; 4.41; 4.41; 4.41; 4.41; 4.41; 4.41; 4.41; 4.41; 4.41; 4.41; 4.41; 4.41; 4.41; 3.2];
      AppIn_LastStoredSOC = 0;
      AppIn_LastStoredCycle = 0;
      AppIn_I2Cerror = false;
      AppIn_LastStoredSOH = 0;
      AppIn_MachineStatus = VDU_MACHINE_STS_E.VDU_SLEEP;
      AppIn_HVMosfetfb = false;
      AppIn_DCDCMosfetfb = false;
      AppIn_PMosfetfb = false;
      AppIn_BMSVltSnsrFail = false;
      AppIn_BattPackTempSnsrFail = false;
      AppIn_VltImbFlt = false;
      AppIn_TempImbWarn = false;
      AppIn_EEPROMSoCWarn15 = false;
    state step_1
      AppIn_OBCwakeup = OBC_E.Wake_Up;
      AppIn_OBCHVIL = true;
    state step_2
      AppIn_BattPackTempSnsrFail = true;
      state step_2_1
        AppIn_PMosfetfb = true;
      state step_2_2
        AppIn_HVMosfetfb = true;
      state step_2_3
        AppIn_PMosfetfb = false;
      (default) -> ChargeSeqG2Fault.step_2.step_2_1
      ChargeSeqG2Fault.step_2.step_2_1 -> ChargeSeqG2Fault.step_2.step_2_2 : [
          | after(0.3,sec)
          | ]
      ChargeSeqG2Fault.step_2.step_2_2 -> ChargeSeqG2Fault.step_2.step_2_3 : [
          | after(0.5,sec)
          | ]
    state step_4
      AppIn_HVMosfetfb = false;
    (default) -> ChargeSeqG2Fault.Run
    ChargeSeqG2Fault.Run -> ChargeSeqG2Fault.step_1 : [
        | after(0.1,sec)
        | ]
    ChargeSeqG2Fault.step_1 -> ChargeSeqG2Fault.step_2 : [
        | after(0.2,sec)
        | ]
    ChargeSeqG2Fault.step_2 -> ChargeSeqG2Fault.step_4 : [
        | after(20,sec)
        | ]
  state ChargeSeq1
    state Run
      %% Initialize data outputs.
      AppIn_HardwiredIgn = false;
      AppIn_OBCwakeup = OBC_E.Sleep;
      AppIn_RTCwakeup = false;
      AppIn_MCUHVIL = false;
      AppIn_OBCHVIL = false;
      AppIn_SoCLEDSW = false;
      AppIn_ChgMode = Charger_Mode_E.OFF;
      AppIn_CVmodeTimer = CV_Mode_Timer_E.Off;
      AppIn_TRerror = false;
      AppIn_TRtimer = false;
      AppIn_G3CommonFlt = false;
      AppIn_G3DischargeFlt = false;
      AppIn_G4T1DischargeFlt = false;
      AppIn_G4T2DischargeFlt = false;
      AppIn_G4CommonFlt = false;
      AppIn_G4ChargeFlt = false;
      AppIn_OBCHeartbeatFail = false;
      AppIn_LoadVolt = 80;
      AppIn_PackVolt = 78;
      AppIn_ActiveDischg = Active_DisChrg_E.Inactive;
      AppIn_BattTemp = [26; 26; 26; 26; 26; 26;];
      AppIn_BattCurrent = 0;
      AppIn_BattVoltages = [4.41; 4.41; 4.41; 4.41; 4.41; 4.41; 4.41; 4.41; 4.41; 4.41; 4.41; 4.41; 4.41; 4.41; 4.41; 4.41; 4.41; 4.41; 4.41; 3.2];
      AppIn_LastStoredSOC = 0;
      AppIn_LastStoredCycle = 0;
      AppIn_I2Cerror = false;
      AppIn_LastStoredSOH = 0;
      AppIn_MachineStatus = VDU_MACHINE_STS_E.VDU_SLEEP;
      AppIn_HVMosfetfb = false;
      AppIn_DCDCMosfetfb = false;
      AppIn_PMosfetfb = false;
      AppIn_BMSVltSnsrFail = false;
      AppIn_BattPackTempSnsrFail = false;
      AppIn_VltImbFlt = false;
      AppIn_TempImbWarn = false;
      AppIn_EEPROMSoCWarn15 = false;
    state step_1
      AppIn_OBCwakeup = OBC_E.Wake_Up;
      AppIn_OBCHVIL = true;
    state step_2
      state step_2_1
        AppIn_PMosfetfb = true;
      state step_2_2
        AppIn_HVMosfetfb = true;
      state step_2_3
        AppIn_PMosfetfb = false;
        AppIn_LoadVolt = 63;
        AppIn_PackVolt = 84;
      (default) -> ChargeSeq1.step_2.step_2_1
      ChargeSeq1.step_2.step_2_1 -> ChargeSeq1.step_2.step_2_2 : [
          | after(0.3,sec)
          | ]
      ChargeSeq1.step_2.step_2_2 -> ChargeSeq1.step_2.step_2_3 : [
          | after(0.5,sec)
          | ]
    state step_4
      AppIn_BattVoltages = [4.41; 4.41; 4.41; 4.41; 4.41; 2.0; 4.41; 4.41; 4.41; 4.41; 4.41; 4.41; 4.41; 4.41; 4.41; 4.41; 4.41; 4.41; 4.41; 3.2];
    (default) -> ChargeSeq1.Run
    ChargeSeq1.Run -> ChargeSeq1.step_1 : [
        | after(0.1,sec)
        | ]
    ChargeSeq1.step_1 -> ChargeSeq1.step_2 : [
        | after(0.2,sec)
        | ]
    ChargeSeq1.step_2 -> ChargeSeq1.step_4 : [
        | after(6,sec)
        | ]
  (default) -> ChargeWhenIgOn [order 1] : [Active_Scenario_index == 1]
  (default) -> DischgWhenIgOn [order 2] : [Active_Scenario_index == 2]
  (default) -> ChargeWhenIgOff [order 3] : [Active_Scenario_index == 3]
  (default) -> ChgToDischgIgOn [order 4] : [Active_Scenario_index == 4]
  (default) -> SleepToStandby [order 5] : [Active_Scenario_index == 5]
  (default) -> DischgToStandby [order 6] : [Active_Scenario_index == 6]
  (default) -> StandbyToDischgIgOn [order 7] : [Active_Scenario_index == 7]
  (default) -> IgOffToOnInCharge [order 8] : [Active_Scenario_index == 8]
  (default) -> IgOnToOffInCharge [order 9] : [Active_Scenario_index == 9]
  (default) -> VehPoweredOff [order 10] : [Active_Scenario_index == 10]
  (default) -> G4T1DischgFlt [order 11] : [Active_Scenario_index == 11]
  (default) -> G4T2DischgFlt [order 12] : [Active_Scenario_index == 12]
  (default) -> G4CommonFlt [order 13] : [Active_Scenario_index == 13]
  (default) -> G4ChargeFlt [order 14] : [Active_Scenario_index == 14]
  (default) -> DischgToChgIgOn [order 15] : [Active_Scenario_index == 15]
  (default) -> FaultToSleep [order 16] : [Active_Scenario_index == 16]
  (default) -> ChgToStandbyIgOn [order 17] : [Active_Scenario_index == 17]
  (default) -> ChgToStandbyIgOff [order 18] : [Active_Scenario_index == 18]
  (default) -> StandbyToChargeIgOn [order 19] : [Active_Scenario_index == 19]
  (default) -> StandbyToChargeIgOff [order 20] : [Active_Scenario_index == 20]
  (default) -> ChgToFltIgOff [order 21] : [Active_Scenario_index == 21]
  (default) -> FltToChgIgOff [order 22] : [Active_Scenario_index == 22]
  (default) -> FltToChgIgOn [order 23] : [Active_Scenario_index == 23]
  (default) -> PrechgVoltFltWhenIgOn [order 24] : [Active_Scenario_index == 24]
  (default) -> PrechgVoltFltWhenIgOff [order 25] : [Active_Scenario_index == 25]
  (default) -> ChargeSequenceIgOff [order 26] : [Active_Scenario_index == 26]
  (default) -> ChargeSequenceIgOn [order 27] : [Active_Scenario_index == 27]
  (default) -> DischgToChargeAndIgOnToOff [order 28] : [Active_Scenario_index == 28]
  (default) -> G4T2DischargeToSleep [order 29] : [Active_Scenario_index == 29]
  (default) -> G4Typ2DischgToSleep [order 30] : [Active_Scenario_index == 30]
  (default) -> G4T1DischargeToSleep [order 31] : [Active_Scenario_index == 31]
  (default) -> G4Typ1DischgToSleep [order 32] : [Active_Scenario_index == 32]
  (default) -> G4CommonToSleep [order 33] : [Active_Scenario_index == 33]
  (default) -> G4CommToSleep [order 34] : [Active_Scenario_index == 34]
  (default) -> G4ChargeToSleep [order 35] : [Active_Scenario_index == 35]
  (default) -> G4ChgToSleep [order 36] : [Active_Scenario_index == 36]
  (default) -> ChgToDischgToChg [order 37] : [Active_Scenario_index == 37]
  (default) -> G4CommFltToChg [order 38] : [Active_Scenario_index == 38]
  (default) -> G4ChgFltToDischg [order 39] : [Active_Scenario_index == 39]
  (default) -> G4T1DischgToG4T2Dischg [order 40] : [Active_Scenario_index == 40]
  (default) -> SleepToCharge [order 41] : [Active_Scenario_index == 41]
  (default) -> SleepToDischarge [order 42] : [Active_Scenario_index == 42]
  (default) -> SleepToChgToSleep [order 43] : [Active_Scenario_index == 43]
  (default) -> SleepToChg [order 44] : [Active_Scenario_index == 44]
  (default) -> SleepToChrg [order 45] : [Active_Scenario_index == 45]
  (default) -> SleepToStbToG3CommFlt [order 46] : [Active_Scenario_index == 46]
  (default) -> SleepToStbToG4CommFlt [order 47] : [Active_Scenario_index == 47]
  (default) -> SleepToStbToG4CommFlt1 [order 48] : [Active_Scenario_index == 48]
  (default) -> SleepToDischgToFlt [order 49] : [Active_Scenario_index == 49]
  (default) -> SleepToDischgToFlt1 [order 50] : [Active_Scenario_index == 50]
  (default) -> SleepToDischgToFlt2 [order 51] : [Active_Scenario_index == 51]
  (default) -> SleepToDischgToFlt3 [order 52] : [Active_Scenario_index == 52]
  (default) -> SleepToChgToFlt [order 53] : [Active_Scenario_index == 53]
  (default) -> SleepToChgToFltToDischg [order 54] : [Active_Scenario_index == 54]
  (default) -> SleepToChgToFltToDischg1 [order 55] : [Active_Scenario_index == 55]
  (default) -> SleepToDischgToFltToChg [order 56] : [Active_Scenario_index == 56]
  (default) -> SleepToDischgToFltToChg1 [order 57] : [Active_Scenario_index == 57]
  (default) -> SleepToDischgToFltToChg2 [order 58] : [Active_Scenario_index == 58]
  (default) -> ChargingSequence [order 59] : [Active_Scenario_index == 59]
  (default) -> ChargeSeq [order 60] : [Active_Scenario_index == 60]
  (default) -> ChargeSeqG2Fault [order 61] : [Active_Scenario_index == 61]
  (default) -> ChargeSeq1 [order 62] : {assert(Active_Scenario_index == 62,'The value of Scenario Parameter ''Active_Scenario_index'' is not valid. Use the index of the scenario to specify it.')}
  data: AppOut_BMSMODE input Enum: BMS_MODE_E size=[1]; AppOut_PrechgMosfetCmd input boolean size=[1]; AppOut_HVMosfetCmd input boolean size=[1]; AppOut_DCDCMosfetCmd input boolean size=[1]; AppOut_PrechgMosfet input Enum: BMS_PMosfet_STS_E size=[1]; AppOut_HVMosfet input Enum: BMS_HVMosfet_STS_E size=[1]; AppOut_DCDCMosfet input Enum: BMS_DCDCMosfet_STS_E size=[1]; AppOut_ASC_Prep_Flag input boolean size=[1]; AppOut_Chrgr_Prep_Flag input boolean size=[1]; AppOut_PrechgVoltFlt input boolean size=[1]; AppOut_ChgModeReq input Enum: Charger_Mode_Req_E size=[1]; AppOut_ChargeVoltageLt input double size=[1]; AppOut_ChargeCurrentLt input double size=[1]; AppOut_DisplaySoC input uint8 size=[1]; AppOut_BatteryCapacity input double size=[1]; AppOut_LowSoCWarn15 input boolean size=[1]; AppOut_LowSoC input boolean size=[1]; AppOut_LowSoCWarn input boolean size=[1]; AppOut_BattPackSOC input double size=[1]; AppOut_LifeCycle input double size=[1]; AppOut_SOH input double size=[1]; AppOut_CurrentCapacity input double size=[1]; AppOut_SOCcc input fixdt('ufix16_Sp01') size=[1]; AppOut_SOCocvavg input fixdt('ufix16_Sp01') size=[1]; AppOut_SOCocvInit input double size=[1]; AppOut_SOCAvgInitial input double size=[1]; AppOut_AvailableEnergy input double size=[1]; AppOut_ChargeCapacity input double size=[1]; AppOut_DischgCurrLimit input double size=[1, 1]; AppOut_Timer30 input double size=[1]; AppOut_BMS_NM_Msg input Enum: BMS_NM_Msg_E size=[1]; AppOut_RegenOverCurrentFlg input boolean size=[1]; AppOut_RegenCurrent input double size=[1, 1]; AppOut_DerateFlg input boolean size=[1]; AppIn_HardwiredIgn output boolean size=[1]; AppIn_OBCwakeup output Enum: OBC_E size=[1]; AppIn_RTCwakeup output boolean size=[1]; AppIn_MCUHVIL output boolean size=[1]; AppIn_OBCHVIL output boolean size=[1]; AppIn_SoCLEDSW output boolean size=[1]; AppIn_ChgMode output Enum: Charger_Mode_E size=[1]; AppIn_CVmodeTimer output Enum: CV_Mode_Timer_E size=[1]; AppIn_TRerror output boolean size=[1]; AppIn_TRtimer output boolean size=[1]; AppIn_G3CommonFlt output boolean size=[1]; AppIn_G3DischargeFlt output boolean size=[1]; AppIn_G4T1DischargeFlt output boolean size=[1]; AppIn_G4T2DischargeFlt output boolean size=[1]; AppIn_G4CommonFlt output boolean size=[1]; AppIn_G4ChargeFlt output boolean size=[1]; AppIn_OBCHeartbeatFail output boolean size=[1]; AppIn_LoadVolt output double size=[1]; AppIn_PackVolt output double size=[1]; AppIn_ActiveDischg output Enum: Active_DisChrg_E size=[1]; AppIn_BattTemp output double size=[6, 1]; AppIn_BattCurrent output double size=[1]; AppIn_BattVoltages output double size=[20, 1]; AppIn_LastStoredSOC output double size=[1]; AppIn_LastStoredCycle output double size=[1]; AppIn_I2Cerror output boolean size=[1]; AppIn_LastStoredSOH output double size=[1]; AppIn_MachineStatus output Enum: VDU_MACHINE_STS_E size=[1]; AppIn_HVMosfetfb output boolean size=[1]; AppIn_DCDCMosfetfb output boolean size=[1]; AppIn_PMosfetfb output boolean size=[1]; AppIn_BMSVltSnsrFail output boolean size=[1]; AppIn_BattPackTempSnsrFail output boolean size=[1]; AppIn_VltImbFlt output boolean size=[1]; AppIn_TempImbWarn output boolean size=[1]; Active_Scenario_index parameter; AppOut_BattTempDerating input; AppOut_BattSoCDerating input; AppIn_EEPROMSoCWarn15 output
